simulink model "tema3b_simscape"  (R2026a)
settings: Solver=ode23t  StopTime=T_sim  MaxStep=2e-6  RelTol=1e-4
values from neighbouring files (symbols this model uses):
  R = u_out/I_out_max    (= 1.25)    [proiect.m]    (also in tema2_simscape.m; tema3.m)
  u_out = 20    [proiect.m]    (also in tema2_simscape.m; tema3.m)
  U_pwm = 5    [tema2_simscape.m]    (also in tema3b.m)
undefined symbols (not defined in the file or in its folder): den_c, num_c
libraries: fl_lib x19, nesl_utility x6, ee_lib x4
settings Model: Creator=Fer Alexandru  LastModifiedBy=Fer Alexandru

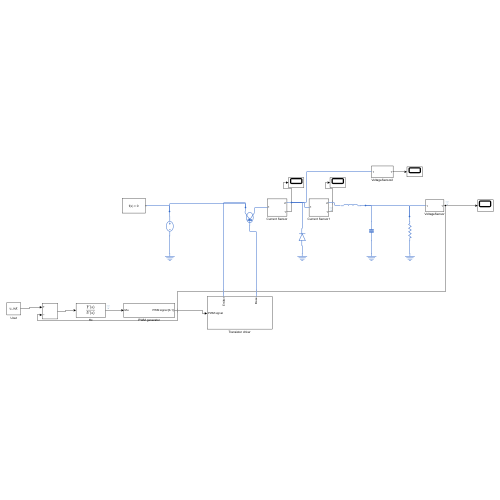
[thumbnail: Simulink's stored preview of the top-level diagram]
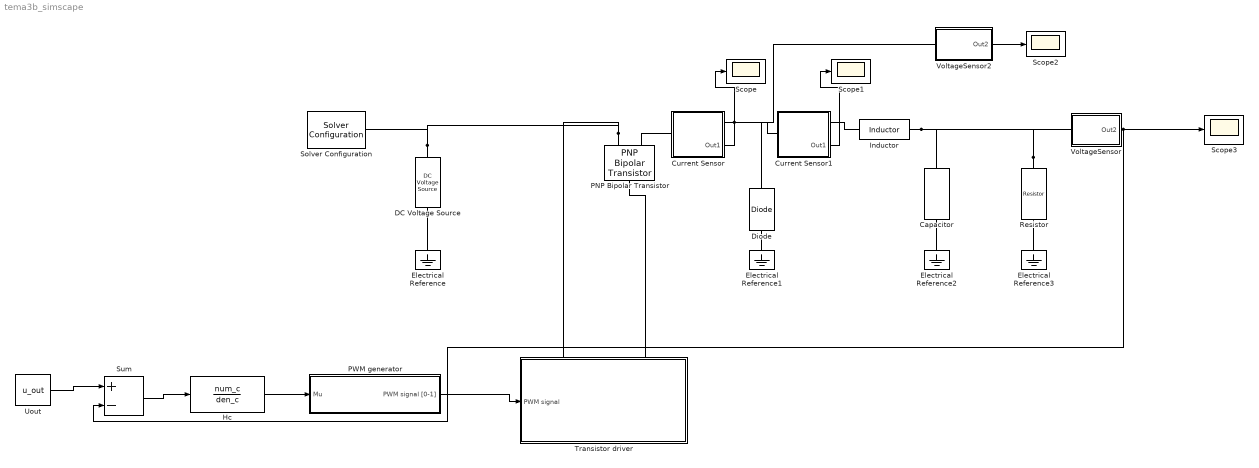
== system tema3b_simscape ==
  Capacitor : ee_lib/Passive/Capacitor  cap_option=ee.enum.passive.capacitor.capOption.const  c=C_nom F  Cvec=[1e-05, 1e-06] F  Vvec=[0, 10] V  CV_table_symmetry=ee.enum.passive.capacitor.tableSymmetry.yes  f_vec=[1, 10] kHz  DFext_vec=[.8, 1.2]  enable_C_tol=ee.enum.toleranceApplication.applyMin  averaging_period=0 s  C_tol=tolC  tol_distribution=ee.enum.toleranceDistribution.uniform  nSigma=4  r=ESR Ohm  g=0 1/Ohm  enable_operating_limits=ee.enum.enable.no  operating_limit_action=ee.enum.passive.reportOpLim.warn  max_working_voltage_range=[-25, 25] V  power_rating=1 W  maxTemperature=85 degC  thermalEnable=false  thermalMass=1 J/K  i_specify=off  i_priority=None  i=0 A  i_nominal_specify=off  i_nominal_value=1  i_nominal_unit=A  v_specify=off  v_priority=None  v=0 V  v_nominal_specify=off  v_nominal_value=1  v_nominal_unit=V  vc_specify=off  vc_priority=High  vc=0 V  vc_nominal_specify=off  vc_nominal_value=1  vc_nominal_unit=V  T_specify=off  T_priority=None  T=298.15 K  T_nominal_specify=off  T_nominal_value=1  T_nominal_unit=K
  Current Sensor : Subsystem
      settings: PortSchema="{\"entries\":[{\"content\":{\"sides\":[{\"content\":{\"connectorIds\":[\"LConn1\"]},\"type\":\"ConnectorPlacement.EquallySpacedRectSide\",\"uuid\":\"879ab8e1-2049-4fb6-a8df-ff1276883f7d\"},{\"content\":{\"connectorIds\":[\"RConn1\",\"Out1\"],\"side\":\"RIGHT\"},\"type\":\"ConnectorPlacement.EquallySpacedRectSide\",\"uuid\":\"0e1e5d09-9c15-402d-9d9c-86393e5954a8\"},{\"content\":{\"side\":\"TOP\"},\"type\":\"ConnectorPlacement.EquallySpacedRectSide\",\"uuid\":\"a34ce212-58b0-488c-a820-7ab63fbdabb5\"}]},\"type\":\"ConnectorPlacement.EquallySpacedConnector\",\"uuid\":\"d04d41d3-98ba-4b02-a4fb-520314011242\"}],\"packageUris\":[\"http://schema.mathworks.com/mf0/Connector/R2020b\"],\"version\":\"1.0\"}"
  Current Sensor1 : Subsystem
      settings: PortSchema="{\"entries\":[{\"content\":{\"sides\":[{\"content\":{\"connectorIds\":[\"LConn1\"]},\"type\":\"ConnectorPlacement.EquallySpacedRectSide\",\"uuid\":\"879ab8e1-2049-4fb6-a8df-ff1276883f7d\"},{\"content\":{\"connectorIds\":[\"RConn1\",\"Out1\"],\"side\":\"RIGHT\"},\"type\":\"ConnectorPlacement.EquallySpacedRectSide\",\"uuid\":\"0e1e5d09-9c15-402d-9d9c-86393e5954a8\"},{\"content\":{\"side\":\"TOP\"},\"type\":\"ConnectorPlacement.EquallySpacedRectSide\",\"uuid\":\"a34ce212-58b0-488c-a820-7ab63fbdabb5\"}]},\"type\":\"ConnectorPlacement.EquallySpacedConnector\",\"uuid\":\"d04d41d3-98ba-4b02-a4fb-520314011242\"}],\"packageUris\":[\"http://schema.mathworks.com/mf0/Connector/R2020b\"],\"version\":\"1.0\"}"
  DC Voltage Source : fl_lib/Electrical/Electrical Sources/DC Voltage Source  v0=u_in V
  Diode : fl_lib/Electrical/Electrical Elements/Diode  Vf=Vf V  Ron=Ron_d Ohm  Goff=1e-8 1/Ohm  i_specify=off  i_priority=None  i=0 A  i_nominal_specify=off  i_nominal_value=1  i_nominal_unit=A  v_specify=off  v_priority=None  v=0 V  v_nominal_specify=off  v_nominal_value=1  v_nominal_unit=V
  Electrical Reference{,1..3} (4 alike) : fl_lib/Electrical/Electrical Elements/Electrical Reference
  Hc : TransferFcn  Numerator=num_c  Denominator=den_c
  Inductor : ee_lib/Passive/Inductor  l=L_nom H  enable_L_tol=ee.enum.toleranceApplication.applyMin  L_tol=tolL  tol_distribution=ee.enum.toleranceDistribution.uniform  nSigma=4  r=DCR Ohm  g=1e-9 1/Ohm  enable_operating_limits=ee.enum.enable.no  operating_limit_action=ee.enum.passive.reportOpLim.warn  max_working_current=1 A  power_rating=1 W  i_L_specify=off  i_L_priority=High  i_L=0 A  i_L_nominal_specify=off  i_L_nominal_value=1  i_L_nominal_unit=A
  PNP Bipolar Transistor : ee_lib/Semiconductors & Converters/PNP Bipolar Transistor  parameterization=1  BF=BF_T1  IS=1e-14 A  VAF=200 V  hfe=BF_T1  hoe=50e-6 1/Ohm  Ic_h=-1 mA  Vce_h=-5 V  V1=-0.55 V  I1=-0.5 mA  BR=1  Tmeas=25 degC  RC=0.01 Ohm  RE=1e-4 Ohm  RB=1 Ohm  C_BC=5 pF  C_BE=5 pF  TF=0 us  TR=0 us  prmDatasheet=1  prmEquCoeff=1  hfe_T2=125  XTB=0  V1_T2=-0.45 V  I1_T2=-0.5 mA  Tmeas2=125 degC  EG=1.11 eV  XTI=3  TdeviceDatasheet=25 degC  TdeviceEquCoeff=25 degC  ec=1  ib_specify=off  ib_priority=None  ib=0 A  ib_nominal_specify=off  ib_nominal_value=1  ib_nominal_unit=A  ic_specify=off  ic_priority=None  ic=0 A  ic_nominal_specify=off  ic_nominal_value=1  ic_nominal_unit=A  vce_specify=off  vce_priority=None  vce=0 V  vce_nominal_specify=off  vce_nominal_value=1  vce_nominal_unit=V  vbe_specify=off  vbe_priority=None  vbe=0 V  vbe_nominal_specify=off  vbe_nominal_value=1  vbe_nominal_unit=V  Qbc_specify=off  Qbc_priority=High  Qbc=0 C  Qbc_nominal_specify=off  Qbc_nominal_value=1  Qbc_nominal_unit=uC  Qbe_specify=off  Qbe_priority=High  Qbe=0 C  Qbe_nominal_specify=off  Qbe_nominal_value=1  Qbe_nominal_unit=uC  thermal_network_parameterization=ee.enum.thermalNetworkTopology.junctionCase  Rth=[0, 10] K/W  Rth_Cauer=[1, 3, 10] K/W  Rth_Foster=[.08, .14, .22, .16] K/W  thermal_mass_parameterization=ee.enum.thermalNetwork.timeconstant  thermal_mass=[0, 1] J/K  thermal_mass_Cauer=[.1, .3, 1] J/K  thermal_mass_Foster=[.001, .005, .05, .5] J/K  thermal_time_constant=[0, 10] s  thermal_time_constant_Cauer=[1, 3, 10] s  thermal_time_constant_Foster=[7e-05, .0007, .01, .08] s  thermal_mass_initial_temperatures=[25, 25] degC  thermal_mass_initial_temperatures_Cauer=[25, 25, 25] degC  Tvec_initial_Foster=[25, 25, 25, 25] degC
  PWM generator : Subsystem
  Resistor : fl_lib/Electrical/Electrical Elements/Resistor  R=R Ohm  i_specify=off  i_priority=None  i=0 A  i_nominal_specify=off  i_nominal_value=1  i_nominal_unit=A  v_specify=off  v_priority=None  v=0 V  v_nominal_specify=off  v_nominal_value=1  v_nominal_unit=V
  Scope{,1..3} (4 alike) : Scope
  Solver Configuration : nesl_utility/Solver Configuration  PhysicalDomain=network_engine_domain  SubClassName=solver  LeftPortType=input  RightPortType=generic  Tones=[]  Harmonics=[]  SimulateNoise=off  Profile=off  UseLocalSampling=off  EnableSwitchedLinearOptims=on  FrequencyDomain=off  UseCCode=off  RelTol=0.001  AbsTol=0.001  MinStep=1e-09  ToWorkspace=off  RevertToSquareIcSolve=off  NumHomotopyIterations=100  PhasorMode=off  PhasorModeNumHarmonics=1  ConsistencySolver=NEWTON_XTOL_AFTER_FTOL  CanonicalOrdering=CANONICAL  OptimizeIntermediates=OPTIMIZED  IndexReductionMethod=DerivativeReplacement  DoDC=off  ResidualTolerance=1e-09  ConsistencyTolSource=GLOBAL  ConsistencyAbsTol=0.001  ConsistencyRelTol=0.001  ConsistencyTolFactor=0.001  UseLocalSolver=off  LocalSolverChoice=NE_BACKWARD_EULER_ADVANCER  ResolveIndetEquations=on  FunctionEvalNumThread=1  LocalSolverSampleTime=0.001  DoFixedCost=off  MaxNonlinIter=3  MaxModeIter=2  ComputeImpulses=off  ImpulseIterations=2  LinearAlgebra=auto  LinearAlgebraNumThread=0  EquationFormulation=NE_TIME_EF  DelaysMemoryBudget=1024  AutomaticFiltering=on  FilteringTimeConstant=0.001  PartitionStorageMethod=AS_NEEDED  PartitionMemoryBudget=1024  PartitionMethod=ROBUST  MultibodyUseLocalSolver=off  MultibodyLocalSolverChoice=ODE1  MultibodyLocalSolverSampleTime=0.001
  Sum : Sum  Inputs=+-
  Transistor driver : Subsystem
      settings: PortSchema="{\"entries\":[{\"content\":{\"sides\":[{\"content\":{\"connectorIds\":[\"In1\"]},\"type\":\"ConnectorPlacement.EquallySpacedRectSide\",\"uuid\":\"f2843adf-4a2d-4dc1-8ed8-7a0d033a9ef4\"},{\"content\":{\"side\":\"RIGHT\"},\"type\":\"ConnectorPlacement.EquallySpacedRectSide\",\"uuid\":\"53271389-a6df-499f-a19b-3cf558d806d4\"},{\"content\":{\"connectorIds\":[\"LConn1\",\"LConn2\"],\"side\":\"TOP\"},\"type\":\"ConnectorPlacement.EquallySpacedRectSide\",\"uuid\":\"0c4fcd1c-45b8-4547-ae44-81f67bad391c\"}]},\"type\":\"ConnectorPlacement.EquallySpacedConnector\",\"uuid\":\"f41e5fa1-c36e-4517-8980-74cbc2e9efc4\"}],\"packageUris\":[\"http://schema.mathworks.com/mf0/Connector/R2020b\"],\"version\":\"1.0\"}"
  Uout : Constant  Value=u_out
  VoltageSensor : Subsystem
  VoltageSensor2 : Subsystem
  wires:
  Uout/1 -> Sum/1
  Sum/1 -> Hc/1
  Hc/1 -> PWM generator/1(Mu)
  VoltageSensor/1(Out2) -> Sum/2, Scope3/1
  PWM generator/1(PWM signal [0-1]) -> Transistor driver/1(PWM signal)
  Current Sensor/1(Out1) -> Scope/1
  Current Sensor1/1(Out1) -> Scope1/1
  VoltageSensor2/1(Out2) -> Scope2/1
  connections:
  DC Voltage Source/LConn1 -- Solver Configuration/RConn1 -- PNP Bipolar Transistor/RConn1 -- Transistor driver/LConn1
  Transistor driver/LConn2 -- PNP Bipolar Transistor/LConn1
  DC Voltage Source/RConn1 -- Electrical Reference/LConn1
  PNP Bipolar Transistor/RConn2 -- Current Sensor/LConn1
  Current Sensor1/LConn1 -- Current Sensor/RConn1 -- Diode/RConn1 -- VoltageSensor2/LConn1
  Diode/LConn1 -- Electrical Reference1/LConn1
  Current Sensor1/RConn1 -- Inductor/LConn1
  Capacitor/LConn1 -- Inductor/RConn1 -- Resistor/LConn1 -- VoltageSensor/LConn1
  Capacitor/RConn1 -- Electrical Reference2/LConn1
  Resistor/RConn1 -- Electrical Reference3/LConn1

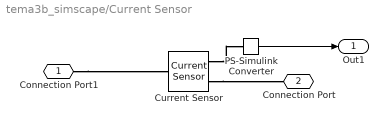
== system tema3b_simscape/Current Sensor ==
  Current Sensor : fl_lib/Electrical/Electrical Sensors/Current Sensor
  PS-Simulink Converter : nesl_utility/PS-Simulink Converter  PhysicalDomain=network_engine_domain  SubClassName=ps_output  LeftPortType=input  RightPortType=output  PseudoPeriodic=off  Frequencies=[]  VectorFormat=inherit  Unit=inherit  AffineConversion=off
  Connection Port1 : PMIOPort  Side=Left
  Connection Port : PMIOPort  Port=2  Side=Right
  Out1 : Outport
  wires:
  PS-Simulink Converter/1 -> Out1/1
  connections:
  Current Sensor/RConn2 -- Connection Port/RConn1
  Current Sensor/RConn1 -- PS-Simulink Converter/LConn1
  Connection Port1/RConn1 -- Current Sensor/LConn1

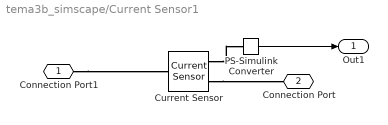
== system tema3b_simscape/Current Sensor1 ==
  Current Sensor : fl_lib/Electrical/Electrical Sensors/Current Sensor
  PS-Simulink Converter : nesl_utility/PS-Simulink Converter  PhysicalDomain=network_engine_domain  SubClassName=ps_output  LeftPortType=input  RightPortType=output  PseudoPeriodic=off  Frequencies=[]  VectorFormat=inherit  Unit=inherit  AffineConversion=off
  Connection Port1 : PMIOPort  Side=Left
  Connection Port : PMIOPort  Port=2  Side=Right
  Out1 : Outport
  wires:
  PS-Simulink Converter/1 -> Out1/1
  connections:
  Current Sensor/RConn2 -- Connection Port/RConn1
  Current Sensor/RConn1 -- PS-Simulink Converter/LConn1
  Connection Port1/RConn1 -- Current Sensor/LConn1

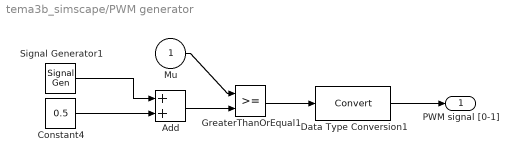
== system tema3b_simscape/PWM generator ==
  Mu : Inport
  Add : Sum
  Constant4 : Constant  Value=0.5
  Data Type Conversion1 : DataTypeConversion  SaturateOnIntegerOverflow=off  RndMeth=Floor
  GreaterThanOrEqual1 : RelationalOperator  OutDataTypeStr=boolean  RndMeth=Simplest  InputSameDT=off
  Signal Generator1 : SignalGenerator  WaveForm=sawtooth  Amplitude=0.5  Frequency=800
  PWM signal [0-1] : Outport
  wires:
  Signal Generator1/1 -> Add/1
  GreaterThanOrEqual1/1 -> Data Type Conversion1/1
  Data Type Conversion1/1 -> PWM signal [0-1]/1
  Constant4/1 -> Add/2
  Add/1 -> GreaterThanOrEqual1/2
  Mu/1 -> GreaterThanOrEqual1/1

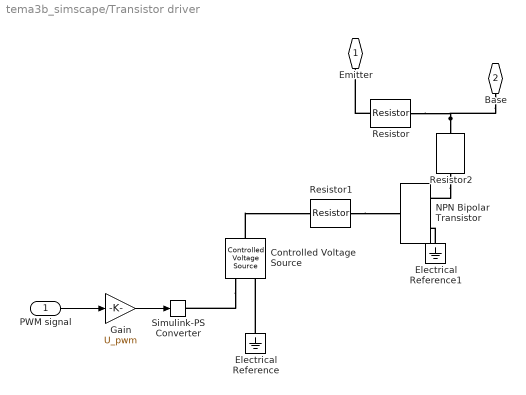
== system tema3b_simscape/Transistor driver ==
  PWM signal : Inport
  Controlled Voltage Source : fl_lib/Electrical/Electrical Sources/Controlled Voltage Source
  Electrical Reference : fl_lib/Electrical/Electrical Elements/Electrical Reference
  Electrical Reference1 : fl_lib/Electrical/Electrical Elements/Electrical Reference
  Gain : Gain  Gain=U_pwm
  NPN Bipolar Transistor : ee_lib/Semiconductors & Converters/NPN Bipolar Transistor  parameterization=1  BF=100  IS=1e-14 A  VAF=200 V  hfe=100  hoe=50e-6 1/Ohm  Ic_h=1 mA  Vce_h=5 V  V1=0.55 V  I1=0.5 mA  BR=1  Tmeas=25 degC  RC=0.01 Ohm  RE=1e-4 Ohm  RB=1 Ohm  C_BC=5 pF  C_BE=5 pF  TF=0 us  TR=0 us  prmDatasheet=1  prmEquCoeff=1  hfe_T2=125  XTB=0  V1_T2=0.45 V  I1_T2=0.5 mA  Tmeas2=125 degC  EG=1.11 eV  XTI=3  TdeviceDatasheet=25 degC  TdeviceEquCoeff=25 degC  ec=1  ib_specify=off  ib_priority=None  ib=0 A  ib_nominal_specify=off  ib_nominal_value=1  ib_nominal_unit=A  ic_specify=off  ic_priority=None  ic=0 A  ic_nominal_specify=off  ic_nominal_value=1  ic_nominal_unit=A  vce_specify=off  vce_priority=None  vce=0 V  vce_nominal_specify=off  vce_nominal_value=1  vce_nominal_unit=V  vbe_specify=off  vbe_priority=None  vbe=0 V  vbe_nominal_specify=off  vbe_nominal_value=1  vbe_nominal_unit=V  Qbc_specify=off  Qbc_priority=High  Qbc=0 C  Qbc_nominal_specify=off  Qbc_nominal_value=1  Qbc_nominal_unit=uC  Qbe_specify=off  Qbe_priority=High  Qbe=0 C  Qbe_nominal_specify=off  Qbe_nominal_value=1  Qbe_nominal_unit=uC  thermal_network_parameterization=ee.enum.thermalNetworkTopology.junctionCase  Rth=[0, 10] K/W  Rth_Cauer=[1, 3, 10] K/W  Rth_Foster=[.08, .14, .22, .16] K/W  thermal_mass_parameterization=ee.enum.thermalNetwork.timeconstant  thermal_mass=[0, 1] J/K  thermal_mass_Cauer=[.1, .3, 1] J/K  thermal_mass_Foster=[.001, .005, .05, .5] J/K  thermal_time_constant=[0, 10] s  thermal_time_constant_Cauer=[1, 3, 10] s  thermal_time_constant_Foster=[7e-05, .0007, .01, .08] s  thermal_mass_initial_temperatures=[25, 25] degC  thermal_mass_initial_temperatures_Cauer=[25, 25, 25] degC  Tvec_initial_Foster=[25, 25, 25, 25] degC
  Resistor : fl_lib/Electrical/Electrical Elements/Resistor  R=1 Ohm  i_specify=off  i_priority=None  i=0 A  i_nominal_specify=off  i_nominal_value=1  i_nominal_unit=A  v_specify=off  v_priority=None  v=0 V  v_nominal_specify=off  v_nominal_value=1  v_nominal_unit=V
  Resistor1 : fl_lib/Electrical/Electrical Elements/Resistor  R=1 Ohm  i_specify=off  i_priority=None  i=0 A  i_nominal_specify=off  i_nominal_value=1  i_nominal_unit=A  v_specify=off  v_priority=None  v=0 V  v_nominal_specify=off  v_nominal_value=1  v_nominal_unit=V
  Resistor2 : fl_lib/Electrical/Electrical Elements/Resistor  R=1 Ohm  i_specify=off  i_priority=None  i=0 A  i_nominal_specify=off  i_nominal_value=1  i_nominal_unit=A  v_specify=off  v_priority=None  v=0 V  v_nominal_specify=off  v_nominal_value=1  v_nominal_unit=V
  Simulink-PS Converter : nesl_utility/Simulink-PS Converter  PhysicalDomain=network_engine_domain  SubClassName=ps_input  LeftPortType=input  RightPortType=output  PseudoPeriodic=off  Frequencies=[]  NoiseDistribution=none  NoiseParameters=[]  Unit=1  AffineConversion=off  FilteringAndDerivatives=provide  SimscapeFilterOrder=1  InputFilterTimeConstant=0.001  UdotUserProvided=0
  Emitter : PMIOPort  Side=Left
  Base : PMIOPort  Port=2  Side=Left
  wires:
  Gain/1 -> Simulink-PS Converter/1
  PWM signal/1 -> Gain/1
  connections:
  Resistor2/RConn1 -- NPN Bipolar Transistor/RConn1
  Controlled Voltage Source/LConn1 -- Resistor1/RConn1
  Electrical Reference/LConn1 -- Controlled Voltage Source/RConn2
  Controlled Voltage Source/RConn1 -- Simulink-PS Converter/RConn1
  Resistor/LConn1 -- Emitter/RConn1
  Resistor2/LConn1 -- Base/RConn1 -- Resistor/RConn1
  Resistor1/LConn1 -- NPN Bipolar Transistor/LConn1
  Electrical Reference1/LConn1 -- NPN Bipolar Transistor/RConn2

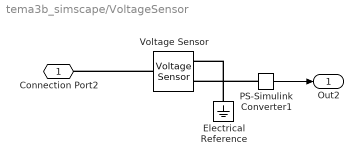
== system tema3b_simscape/VoltageSensor ==
  Electrical Reference : fl_lib/Electrical/Electrical Elements/Electrical Reference
  PS-Simulink Converter1 : nesl_utility/PS-Simulink Converter  PhysicalDomain=network_engine_domain  SubClassName=ps_output  LeftPortType=input  RightPortType=output  PseudoPeriodic=off  Frequencies=[]  VectorFormat=inherit  Unit=inherit  AffineConversion=off
  Voltage Sensor : fl_lib/Electrical/Electrical Sensors/Voltage Sensor
  Connection Port2 : PMIOPort  Side=Left
  Out2 : Outport
  wires:
  PS-Simulink Converter1/1 -> Out2/1
  connections:
  Electrical Reference/LConn1 -- Voltage Sensor/RConn2
  PS-Simulink Converter1/LConn1 -- Voltage Sensor/RConn1
  Voltage Sensor/LConn1 -- Connection Port2/RConn1

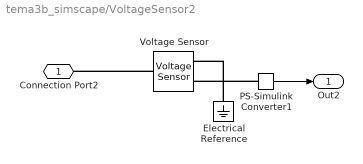
== system tema3b_simscape/VoltageSensor2 ==
  Electrical Reference : fl_lib/Electrical/Electrical Elements/Electrical Reference
  PS-Simulink Converter1 : nesl_utility/PS-Simulink Converter  PhysicalDomain=network_engine_domain  SubClassName=ps_output  LeftPortType=input  RightPortType=output  PseudoPeriodic=off  Frequencies=[]  VectorFormat=inherit  Unit=inherit  AffineConversion=off
  Voltage Sensor : fl_lib/Electrical/Electrical Sensors/Voltage Sensor
  Connection Port2 : PMIOPort  Side=Left
  Out2 : Outport
  wires:
  PS-Simulink Converter1/1 -> Out2/1
  connections:
  Electrical Reference/LConn1 -- Voltage Sensor/RConn2
  PS-Simulink Converter1/LConn1 -- Voltage Sensor/RConn1
  Voltage Sensor/LConn1 -- Connection Port2/RConn1
